simulink model "ejemplo_balancin"  (R2022b)
settings: Solver=ode4  StartTime=0.0  StopTime=10  FixedStep=Tm/4  RelTol=1e-3
InitFcn:
  | init_ejemplo
values from neighbouring files (symbols this model uses):
  Ap = [0 1; 0 0]    [init_ejemplo.m]
  Bp = [0; l/J]    [init_ejemplo.m]
  Cp = eye(2)    [init_ejemplo.m]
  Dp = [0; 0]    [init_ejemplo.m]
  Gm_den = [1 268.5 33190]    [init_ejemplo.m]
  Gm_num = 8630    [init_ejemplo.m]
  Kth = 4    [init_ejemplo.m]
  ref = deg2rad(10)    [init_ejemplo.m]
  Tbase = 0.10    (= 0.1)    [init_ejemplo.m]
  Tm = 0.5e-3    (= 0.0005)    [init_ejemplo.m]
  umax = 0.08    [init_ejemplo.m]
  wmax = deg2rad(120)    [init_ejemplo.m]
undefined symbols (not defined in the file or in its folder): ControlDer, ControlPI, Mixer
settings Model: Creator=herna  LastModifiedBy=herna

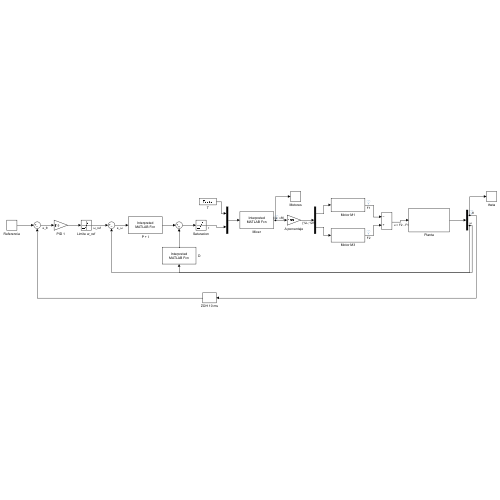
[thumbnail: Simulink's stored preview of the top-level diagram]
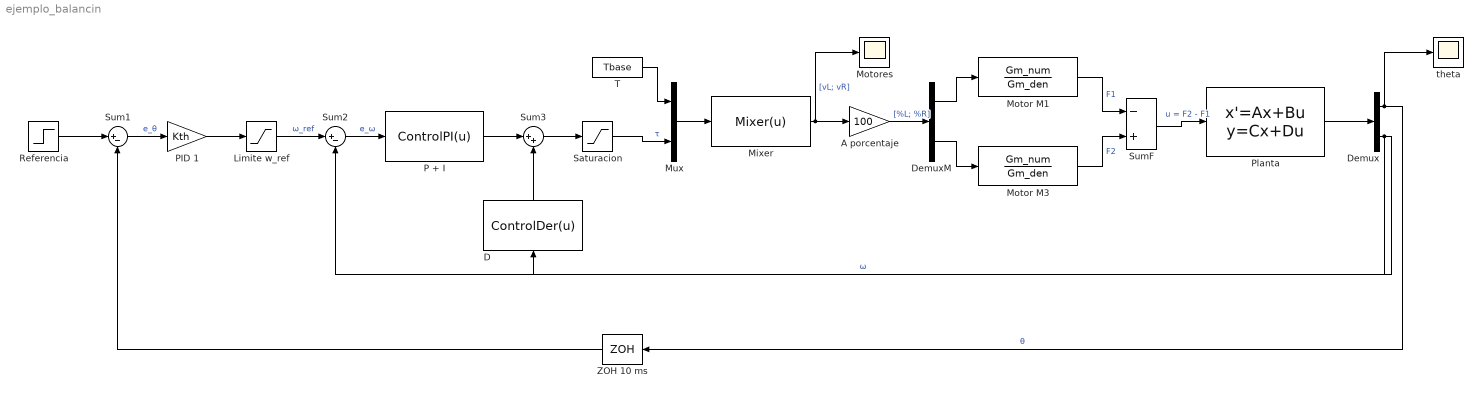
== system ejemplo_balancin ==
  A porcentaje : Gain  Gain=100
  D : MATLABFcn  MATLABFcn=ControlDer(u)  OutputDimensions=1  SampleTime=Tm
  Demux : Demux  Outputs=2
  DemuxM : Demux  Outputs=2
  Limite w_ref : Saturate  UpperLimit=wmax  LowerLimit=-wmax
  Mixer : MATLABFcn  MATLABFcn=Mixer(u)  OutputDimensions=2
  Motor M1 : TransferFcn  Numerator=Gm_num  Denominator=Gm_den
  Motor M3 : TransferFcn  Numerator=Gm_num  Denominator=Gm_den
  Motores : Scope
  Mux : Mux  Inputs=2
  P + I : MATLABFcn  MATLABFcn=ControlPI(u)  OutputDimensions=1  SampleTime=Tm
  PID 1 : Gain  Gain=Kth
  Planta : StateSpace  A=Ap  B=Bp  C=Cp  D=Dp  InitialCondition=[0;0]
  Referencia : Step  Time=0.5  After=ref  SampleTime=0
  Saturacion : Saturate  UpperLimit=umax  LowerLimit=-umax
  Sum1 : Sum  Inputs=|+-
  Sum2 : Sum  Inputs=|+-
  Sum3 : Sum  Inputs=|++
  SumF : Sum  Inputs=-+
  T : Constant  Value=Tbase
  ZOH 10 ms : ZeroOrderHold  SampleTime=0.01
  theta : Scope
  wires:
  Referencia/1 -> Sum1/1
  Sum1/1 -> PID 1/1  "e_θ"
  PID 1/1 -> Limite w_ref/1
  Limite w_ref/1 -> Sum2/1  "ω_ref"
  Sum2/1 -> P + I/1  "e_ω"
  P + I/1 -> Sum3/1
  D/1 -> Sum3/2
  Sum3/1 -> Saturacion/1
  T/1 -> Mux/1
  Saturacion/1 -> Mux/2  "τ"
  Mux/1 -> Mixer/1
  Mixer/1 -> A porcentaje/1, Motores/1  "[vL; vR]"
  A porcentaje/1 -> DemuxM/1  "[%L; %R]"
  DemuxM/1 -> Motor M1/1
  DemuxM/2 -> Motor M3/1
  Motor M1/1 -> SumF/1  "F1"
  Motor M3/1 -> SumF/2  "F2"
  SumF/1 -> Planta/1  "u = F2 - F1"
  Planta/1 -> Demux/1
  Demux/1 -> ZOH 10 ms/1, theta/1  "θ"
  ZOH 10 ms/1 -> Sum1/2
  Demux/2 -> Sum2/2, D/1  "ω"
